simulink model "SensoSpoon_Analytic"  (R2026a)
settings: Solver=ode15s  StopTime=6  MaxStep=.001  RelTol=1e-5  AbsTol=1e-7
model workspace (MAT data in the model file):
  B(1).mass = 0.00253187337457
  B(1).com = [0.000428308261577; -3.33592024592e-19; -1.28078157724e-20]
  B(1).inertia = [7.38028719368e-08  -3.07478426256e-25  -1.32817521062e-25; -3.07478426256e-25  1.0653311692e-08  -5.88805898006e-25; -1.32817521062e-25  -5.88805898006e-25  7.14205635889e-08]
  B(2).mass = 0.043143480036
  B(2).com = [-0.0486280291057; 4.76311480628e-08; -0.0069963183131]
  B(2).inertia = [4.11170784507e-06  8.58555120438e-12  -4.48824336546e-06; 8.58555120438e-12  4.48215975922e-05  4.94803369061e-11; -4.48824336546e-06  4.94803369061e-11  4.62680338807e-05]
  B(3).mass = 0.011
  B(3).com = [0.049; -0.005; 0.006]
  B(3).inertia = [1.98e-07  0  0; 0  2.31e-07  0; 0  0  2.31e-07]
  B(4).mass = 0.0127643184343
  B(4).com = [0.0761622058383; 0.005; 0.006]
  B(4).inertia = [1.99984858239e-07  0  0; 0  2.24509835442e-06  0; 0  0  2.24509835442e-06]
  B(5).mass = 0.000712000026889
  B(5).com = [0; 0; 0]
  B(5).inertia = [3.56000013445e-10  0  0; 0  5.02701685652e-08  0; 0  0  5.02701685652e-08]
  B(6).mass = 0.000712000026889
  B(6).com = [0; 0; 0]
  B(6).inertia = [3.56000013445e-10  0  0; 0  5.02701685652e-08  0; 0  0  5.02701685652e-08]
  H.revision = 'RCFlex_curved_neck_v17'
  H.total_length_mm = 271
  H.handle_mm = [168 30 24]
  H.bowl_mm = [62 40 12]
  H.bowl_tip_x_mm = -103
  H.bowl_widest_station_mm = 37.2
  H.bowl_front_width_mm = 28
  H.bowl_front_station_mm = 10.6338862458
  H.bowl_connection_width_mm = 10
  H.bowl_bottom_thickness_mm = 1.8
  H.bowl_measurement_x_mm = -65.8
  H.bowl_rim_z_mm = -4
  H.neck_length_mm = 31
  H.gimbal_mm = [25 33 19]
  H.pushrod_diameter_mm = 2
  H.physical_travel_deg = 15
  H.grip_x_mm = 65
  H.remote_center_x_mm = NaN
  H.equivalent_center_x_mm = 0
  H.shell_wall_mm = 1.4
  H.shell_x_mm = [0 18 35 55 80 100 130 150 160 168]
  H.shell_y_scale = [1.4 1.33333333333 1.2 1.1 1.08666666667 1.10666666667 1.14666666667 1.08666666667 0.8 0.133333333333]
  H.shell_z_scale = [1.75 1.66666666667 1.48333333333 1.16666666667 1.125 1.16666666667 1.25 1.16666666667 0.916666666667 0.166666666667]
  H.shell_center_z_mm = [0 0 1.5 4 6 6 6 6 6 6]
  H.ball_outer_radius_mm = 17
  H.ball_inner_radius_mm = 16.2
  H.ball_x_limits_mm = [-15.5 -3]
  H.bezel_outer_radius_mm = 21
  H.bezel_inner_radius_mm = 19.8
  H.bezel_x_limits_mm = [-16 0]
  H.front_cap_x_mm = 18
  H.front_rod_windows_mm = [-6.5  -2  9  18; 6.5  -2  9  18]
  H.bowl_wall_mm = 1.2
  H.vca_length_mm = 23.9
  H.vca_diameter_mm = 15.9
  H.vca_centers_mm = [55.5  -5  6; 87.5  5  6]
  H.vca_stroke_mm = 6.35
  H.vca_force_peak_N = 4.6
  H.vca_force_cont_N = 1.5
  H.vca_force_constant_N_A = 1.5
  H.steel_E_Pa = 200000000000
  H.flexure_pivot_parts = {'C-Flex B-10 x2 (pitch)', 'C-Flex D-10 x1 (roll)'}
  H.flexure_stiffness_Nm_rad = [0.00517884308057; 0.0116523969313]
  H.flexure_stiffness_tolerance = 0.1
  H.flexure_damping_Nms_rad = 0.0002
  H.flexure_cubic_ratio = 0
  H.fs = 1000
  H.duration = 20
  H.link.pivot = [0.012  0.012; -0.005  0.005; 0.0075  0.0075]
  H.link.mode = 'direct'
  H.link.attachment = [0.006  0.006; -0.0085  0.0085; -0.01  -0.01]
  H.link.slider_x = [0.03 0.03]
  H.link.slider_z = 0.006
  H.link.input_length = [0.0290559804515 0.0290559804515]
  H.link.output_length = 0
  H.coil_R_ohm = 4.6
  H.coil_L_H = 0.0008
  H.bus_voltage_V = 7.4
  H.current_limit_A = 1.5
  H.coil_alpha_K = 0.00393
  H.coil_mass_kg = 0.011
  H.motor_body_mass_kg = 0.017
  H.coil_continuous_power_W = 4.4
  H.shaft_side_load_N = 2.2
  H.driver_R_ohm = 0.7
  H.driver_pwm_hz = 20000
  H.driver_min_voltage_V = 4.5
  H.battery_capacity_Ah = 0.4
  H.battery_R_ohm = 0.15
  H.battery_mass_kg = 0.018
  H.battery_mm = [41 20 13]
  H.motor_part = 'Moticont GVCM-016-019-01M'
  H.driver_part = 'TI DRV8876PWPR'
  H.guide_friction_N = 0.03
  H.guide_viscous_Ns_m = 0.03
  H.imu_part = 'Bosch BMI270'
  H.imu_gyro_noise_dps_sqrtHz = 0.007
  H.imu_acc_noise_g_sqrtHz = 0.00016
  H.imu_gyro_offset_dps = 0.5
  H.imu_rate_hz = 800
  H.ambient_C = 25
  H.thermal_capacity_J_K = 8
  H.thermal_resistance_K_W = 18
  H.stop_stiffness_Nm_rad = 8
  H.stop_damping_Nms_rad = 0.025
  H.slider_stop_N_m = 10000
  H.slider_stop_Ns_m = 2
  H.food_mass_kg = 0.005
  base_motion = timeseries
  base_motion.Name = 'unnamed'
  base_motion.DataInfo = tsdata.datametadata
  base_motion.DataInfo.Interpolation = tsdata.interpolation
  base_motion.DataInfo.Interpolation.Fhandle : function handle (value not decoded)
  base_motion.DataInfo.Interpolation.Name = 'linear'
  base_motion.TimeInfo = tsdata.timemetadata
  base_motion.TimeInfo.Length = 6001
  base_motion.TimeInfo.DuplicateTimes = 0
  base_motion.TimeInfo.Time_ = [0 0.001 0.002 0.003 0.004 0.005 0.006 0.007 0.008 0.009 0.01 0.011 ... (6001 elements, 6001x1)]
  base_motion.TimeInfo.Initialized = 1
  base_motion.QualityInfo = tsdata.qualmetadata
  base_motion.Data_ = [0 0 0 0 0 0 0 0 0 0 0 0 ... (90015 elements, 6001x15)]
  mode = 'voltage'
  voltage_command = timeseries
  voltage_command.Name = 'unnamed'
  voltage_command.DataInfo = tsdata.datametadata
  voltage_command.DataInfo.Interpolation = tsdata.interpolation
  voltage_command.DataInfo.Interpolation.Fhandle : function handle (value not decoded)
  voltage_command.DataInfo.Interpolation.Name = 'linear'
  voltage_command.TimeInfo = tsdata.timemetadata
  voltage_command.TimeInfo.Length = 6001
  voltage_command.TimeInfo.DuplicateTimes = 0
  voltage_command.TimeInfo.Time_ = [0 0.001 0.002 0.003 0.004 0.005 0.006 0.007 0.008 0.009 0.01 0.011 ... (6001 elements, 6001x1)]
  voltage_command.TimeInfo.Initialized = 1
  voltage_command.QualityInfo = tsdata.qualmetadata
  voltage_command.Data_ = [0 0 0 0 0 0 0 0 0 0 0 0 ... (12002 elements, 6001x2)]
settings Model: Creator=tomli  LastModifiedBy=Aditya

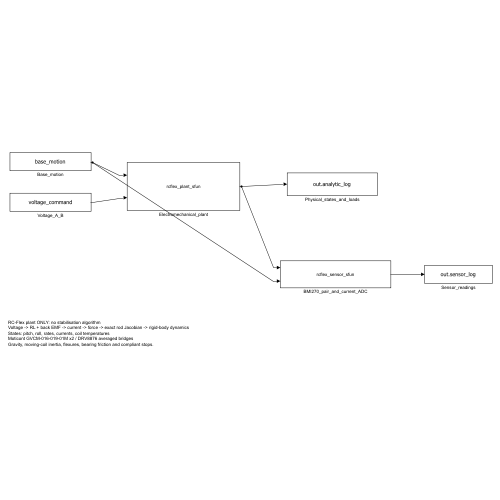
[thumbnail: Simulink's stored preview of the top-level diagram]
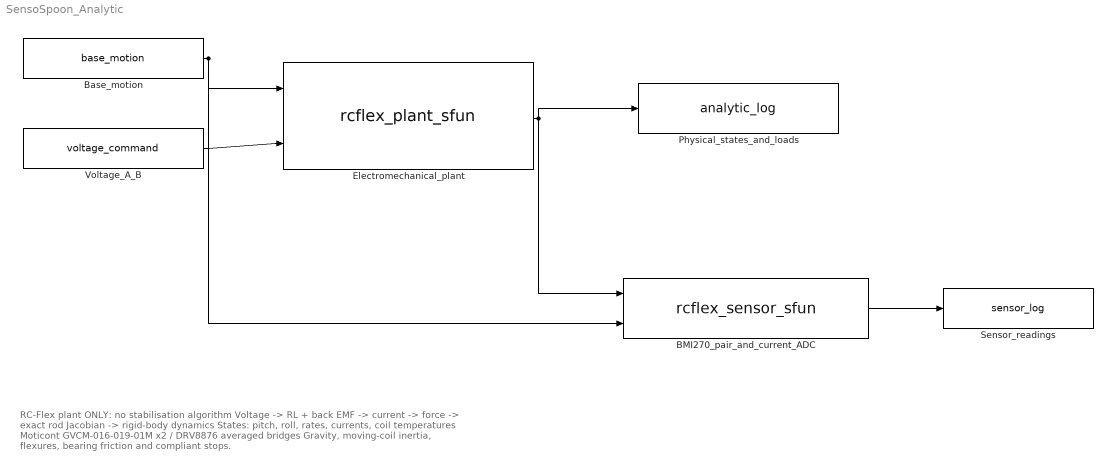
== system SensoSpoon_Analytic ==
  note: RC-Flex plant ONLY: no stabilisation algorithm
      | Voltage -> RL + back EMF -> current -> force -> exact rod Jacobian -> rigid-body dynamics
      | States: pitch, roll, rates, currents, coil temperatures
      | Moticont GVCM-016-019-01M x2 / DRV8876 averaged bridges
      | Gravity, moving-coil inertia, flexures, bearing friction and compliant stops.
  BMI270_pair_and_current_ADC : M-S-Function  FunctionName=rcflex_sensor_sfun  Parameters=H
  Base_motion : FromWorkspace  VariableName=base_motion
  Electromechanical_plant : M-S-Function  FunctionName=rcflex_plant_sfun  Parameters=H,B,mode
  Physical_states_and_loads : ToWorkspace  VariableName=analytic_log  SaveFormat=Timeseries  SampleTime=-1
  Sensor_readings : ToWorkspace  VariableName=sensor_log  SaveFormat=Timeseries  SampleTime=-1
  Voltage_A_B : FromWorkspace  VariableName=voltage_command
  wires:
  Base_motion/1 -> Electromechanical_plant/1, BMI270_pair_and_current_ADC/2
  Voltage_A_B/1 -> Electromechanical_plant/2
  Electromechanical_plant/1 -> Physical_states_and_loads/1, BMI270_pair_and_current_ADC/1
  BMI270_pair_and_current_ADC/1 -> Sensor_readings/1
